simulink model "twin_numerico"  (R2024b)
settings: Solver=ode4  StartTime=0.0  StopTime=20  FixedStep=2e-4  RelTol=1e-3
InitFcn:
  | parameters_charlton;
  | parameters_chamber1d;
  | parameters_ferreira;
  | KT = 1.44; Tmax = KT*Tmax;
  | Emax = 1.40;
  | LAP = 8.50;
undefined symbols (not defined in the file): AP_0, C3, Emin, Ferreira_LV, L, MCL_vascular_lib, P_venous, R1, R2, R3, R4, S_abdominal, S_lower, S_upper, tc, V0, z1_0
settings Model: Creator=sammy  LastModifiedBy=sammy

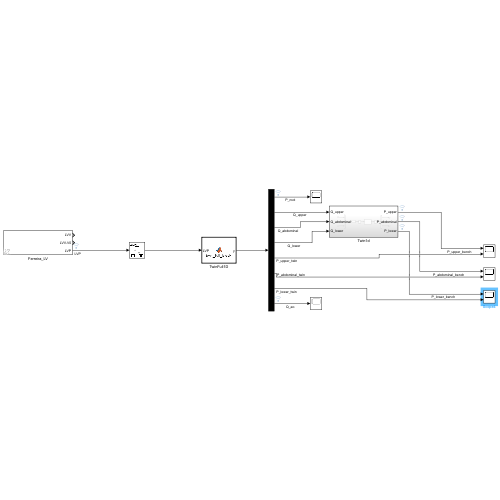
[thumbnail: Simulink's stored preview of the top-level diagram]
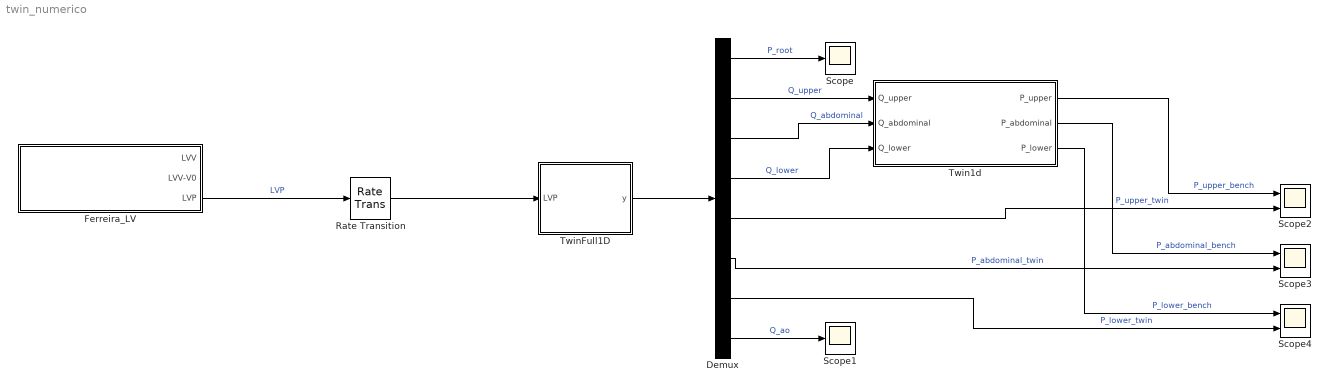
== system twin_numerico ==
  Demux : Demux  Outputs=8
  Ferreira_LV : Subsystem  AncestorBlock=MCL_vascular_lib/Ferreira_LV
  Rate Transition : RateTransition  OutPortSampleTime=1e-3
  Scope : Scope
  Scope1 : Scope
  Scope2 : Scope  NumInputPorts=2
  Scope3 : Scope  NumInputPorts=2
  Scope4 : Scope  NumInputPorts=2
  Twin1d : Subsystem
  TwinFull1D : MATLAB Function  TreatAsAtomicUnit=on
  wires:
  Ferreira_LV/3(LVP) -> Rate Transition/1  "LVP"
  Rate Transition/1 -> TwinFull1D/1(LVP)
  TwinFull1D/1(y) -> Demux/1
  Demux/1 -> Scope/1  "P_root"
  Demux/8 -> Scope1/1  "Q_ao"
  Demux/2 -> Twin1d/1(Q_upper)  "Q_upper"
  Demux/3 -> Twin1d/2(Q_abdominal)  "Q_abdominal"
  Demux/4 -> Twin1d/3(Q_lower)  "Q_lower"
  Demux/5 -> Scope2/2  "P_upper_twin"
  Demux/6 -> Scope3/2  "P_abdominal_twin"
  Demux/7 -> Scope4/2  "P_lower_twin"
  Twin1d/1(P_upper) -> Scope2/1  "P_upper_bench"
  Twin1d/2(P_abdominal) -> Scope3/1  "P_abdominal_bench"
  Twin1d/3(P_lower) -> Scope4/1  "P_lower_bench"

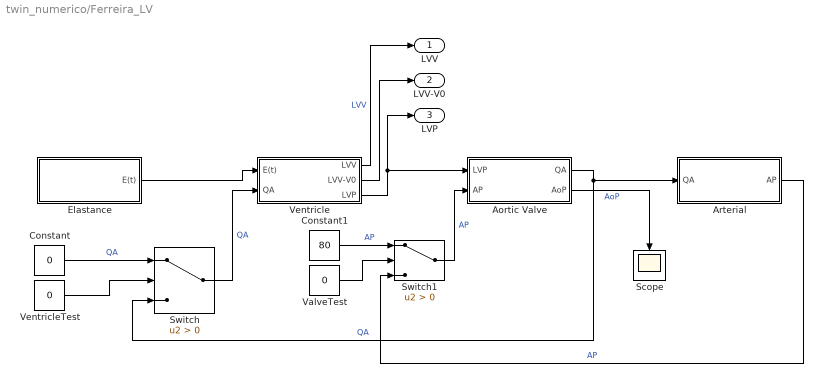
== system twin_numerico/Ferreira_LV ==
  Aortic Valve : Subsystem
  Arterial : Subsystem
  Constant : Constant  Value=0
  Constant1 : Constant  Value=80
  Elastance : Subsystem
  Scope : Scope
  Switch : Switch  Criteria=u2 > Threshold  SaturateOnIntegerOverflow=off  InputSameDT=off
  Switch1 : Switch  Criteria=u2 > Threshold  SaturateOnIntegerOverflow=off  InputSameDT=off
  ValveTest : Constant  Value=0
  Ventricle : Subsystem
  VentricleTest : Constant  Value=0
  LVV : Outport
  LVV-V0 : Outport  Port=2
  LVP : Outport  Port=3
  wires:
  VentricleTest/1 -> Switch/2
  Aortic Valve/1(QA) -> Arterial/1(QA), Switch/3  "QA"
  Ventricle/2(LVV-V0) -> LVV-V0/1
  Elastance/1(E(t)) -> Ventricle/1(E(t))
  Constant/1 -> Switch/1  "QA"
  Constant1/1 -> Switch1/1  "AP"
  Ventricle/3(LVP) -> LVP/1, Aortic Valve/1(LVP)
  Arterial/1(AP) -> Switch1/3  "AP"
  Switch/1 -> Ventricle/2(QA)  "QA"
  ValveTest/1 -> Switch1/2
  Switch1/1 -> Aortic Valve/2(AP)  "AP"
  Ventricle/1(LVV) -> LVV/1  "LVV"
  Aortic Valve/2(AoP) -> Scope/1  "AoP"

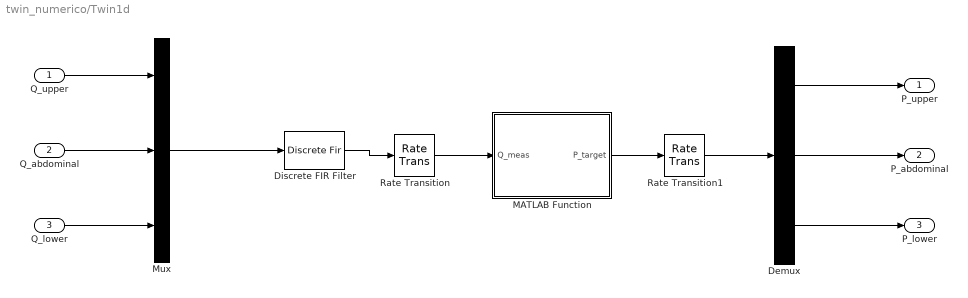
== system twin_numerico/Twin1d ==
  Q_upper : Inport
  Q_abdominal : Inport  Port=2
  Q_lower : Inport  Port=3
  Demux : Demux  Outputs=3
  Discrete FIR Filter : DiscreteFir  Coefficients=ones(1,5)/5
  MATLAB Function : MATLAB Function  TreatAsAtomicUnit=on
  Mux : Mux  Inputs=3
  Rate Transition : RateTransition  OutPortSampleTime=1e-3
  Rate Transition1 : RateTransition  OutPortSampleTime=2e-4
  P_upper : Outport
  P_abdominal : Outport  Port=2
  P_lower : Outport  Port=3
  wires:
  Q_upper/1 -> Mux/1
  Q_abdominal/1 -> Mux/2
  Q_lower/1 -> Mux/3
  Mux/1 -> Discrete FIR Filter/1
  Discrete FIR Filter/1 -> Rate Transition/1
  Rate Transition/1 -> MATLAB Function/1(Q_meas)
  MATLAB Function/1(P_target) -> Rate Transition1/1
  Rate Transition1/1 -> Demux/1
  Demux/1 -> P_upper/1
  Demux/2 -> P_abdominal/1
  Demux/3 -> P_lower/1

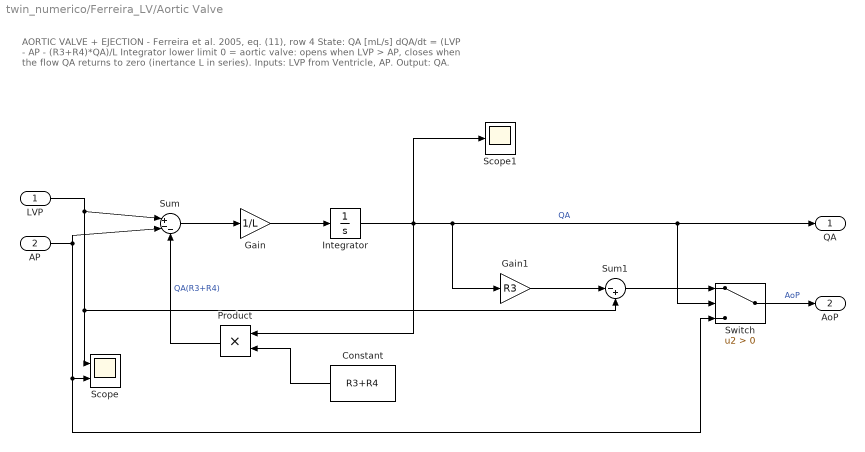
== system twin_numerico/Ferreira_LV/Aortic Valve ==
  note: AORTIC VALVE + EJECTION - Ferreira et al. 2005, eq. (11), row 4
      | State: QA [mL/s] dQA/dt = (LVP - AP - (R3+R4)*QA)/L
      | Integrator lower limit 0 = aortic valve: opens when LVP > AP, closes when the flow QA returns to zero (inertance L in series).
      | Inputs: LVP from Ventricle, AP. Output: QA.
  LVP : Inport
  AP : Inport  Port=2
  Constant : Constant  Value=R3+R4
  Gain : Gain  Gain=1/L
  Gain1 : Gain  Gain=R3
  Integrator : Integrator  LimitOutput=on  LowerSaturationLimit=0
  Product : Product
  Scope : Scope  NumInputPorts=2
  Scope1 : Scope
  Sum : Sum  Inputs=|+--
  Sum1 : Sum  Inputs=|-+
  Switch : Switch  Criteria=u2 > Threshold  SaturateOnIntegerOverflow=off  InputSameDT=off
  QA : Outport
  AoP : Outport  Port=2
  wires:
  LVP/1 -> Sum1/2, Scope/1, Sum/1
  AP/1 -> Switch/3, Scope/2, Sum/2
  Integrator/1 -> Scope1/1, Gain1/1, Switch/2, QA/1, Product/1  "QA"
  Constant/1 -> Product/2
  Product/1 -> Sum/3  "QA(R3+R4)"
  Sum/1 -> Gain/1
  Gain/1 -> Integrator/1
  Gain1/1 -> Sum1/1
  Sum1/1 -> Switch/1
  Switch/1 -> AoP/1  "AoP"

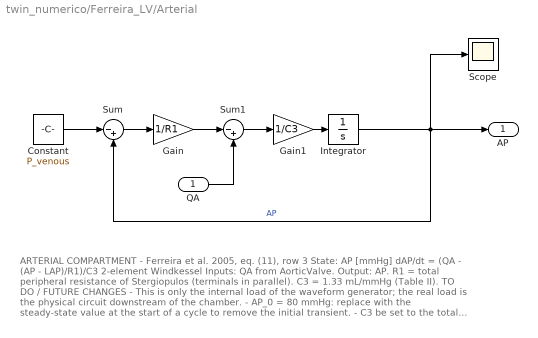
== system twin_numerico/Ferreira_LV/Arterial ==
  note: ARTERIAL COMPARTMENT - Ferreira et al. 2005, eq. (11), row 3
      | State: AP [mmHg] dAP/dt = (QA - (AP - LAP)/R1)/C3 2-element Windkessel
      | Inputs: QA from AorticValve. Output: AP. R1 = total peripheral resistance of Stergiopulos (terminals in parallel). C3 = 1.33 mL/mmHg (Table II).
      | TO DO / FUTURE CHANGES
      | - This is only the internal load of the waveform generator; the real load is the physical circuit downstream of the chamber.
      | - AP_0 = 80 mmHg: replace with the steady-state value at the start of a cycle to remove the initial transient.
      | - C3 be set to the total compliance of the Stergiopulos model for consistency with R1
  QA : Inport
  Constant : Constant  Value=P_venous
  Gain : Gain  Gain=1/R1
  Gain1 : Gain  Gain=1/C3
  Integrator : Integrator  InitialCondition=AP_0
  Scope : Scope
  Sum : Sum  Inputs=|-+
  Sum1 : Sum  Inputs=|-+
  AP : Outport
  wires:
  Constant/1 -> Sum/1
  Integrator/1 -> Scope/1, AP/1, Sum/2  "AP"
  Sum/1 -> Gain/1
  Gain/1 -> Sum1/1
  QA/1 -> Sum1/2
  Sum1/1 -> Gain1/1
  Gain1/1 -> Integrator/1

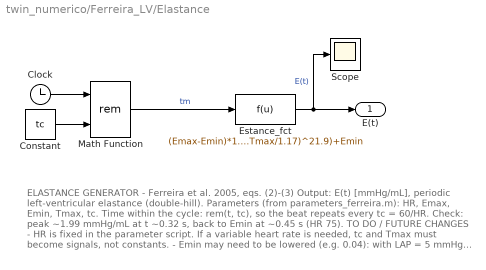
== system twin_numerico/Ferreira_LV/Elastance ==
  note: ELASTANCE GENERATOR - Ferreira et al. 2005, eqs. (2)-(3)
      | Output: E(t) [mmHg/mL], periodic left-ventricular elastance (double-hill).
      | Parameters (from parameters_ferreira.m):
      | HR, Emax, Emin, Tmax, tc.
      | Time within the cycle: rem(t, tc), so the beat repeats every tc = 60/HR.
      | Check: peak ~1.99 mmHg/mL at t ~0.32 s, back to Emin at ~0.45 s (HR 75).
      | TO DO / FUTURE CHANGES
      | - HR is fixed in the parameter script. If a variable heart rate is needed, tc and Tmax must become signals, not constants.
      | - Emin may need to be lowered (e.g. 0.04): with LAP = 5 mmHg the ventricle fills only to z1 = LAP/Emin ~ 83 mL (low stroke volume).
  Clock : Clock
  Constant : Constant  Value=tc
  Estance_fct : Fcn  Expr=(Emax-Emin)*1.55*((u/Tmax/0.7)^1.9/(1+(u/Tmax/0.7)^1.9))/(1+(u/Tmax/1.17)^21.9)+Emin
  Math Function : Math  Operator=rem
  Scope : Scope
  E(t) : Outport
  wires:
  Clock/1 -> Math Function/1
  Math Function/1 -> Estance_fct/1  "tm"
  Constant/1 -> Math Function/2
  Estance_fct/1 -> Scope/1, E(t)/1  "E(t)"

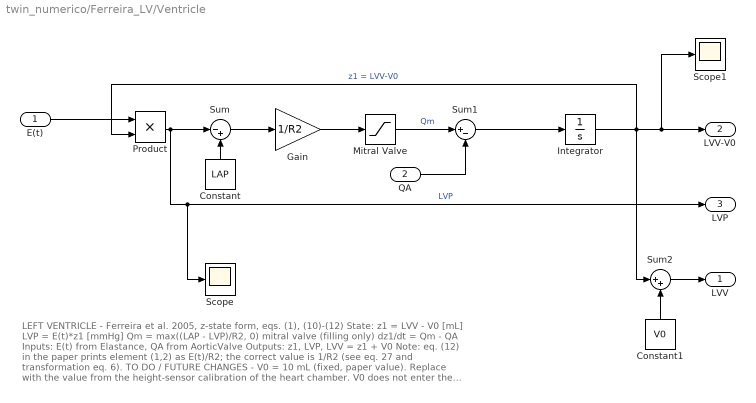
== system twin_numerico/Ferreira_LV/Ventricle ==
  note: LEFT VENTRICLE - Ferreira et al. 2005, z-state form, eqs. (1), (10)-(12)
      | State: z1 = LVV - V0 [mL] LVP = E(t)*z1 [mmHg] Qm = max((LAP - LVP)/R2, 0) mitral valve (filling only) dz1/dt = Qm - QA
      | Inputs: E(t) from Elastance, QA from AorticValve
      | Outputs: z1, LVP, LVV = z1 + V0
      | Note: eq. (12) in the paper prints element (1,2) as E(t)/R2; the correct value is 1/R2 (see eq. 27 and transformation eq. 6).
      | TO DO / FUTURE CHANGES
      | - V0 = 10 mL (fixed, paper value). Replace with the value from the height-sensor calibration of the heart chamber. V0 does not enter the dynamics, only the output LVV = z1 + V0. - LAP = P_venous (5 mmHg, constant), taken from parameters_stergiopulos.m. . - The output used by the physical chamber is the volume (LVV or z1); the conversion to pressure / chamber command is done outside this block.
  E(t) : Inport
  QA : Inport  Port=2
  Constant : Constant  Value=LAP
  Constant1 : Constant  Value=V0
  Gain : Gain  Gain=1/R2
  Integrator : Integrator  InitialCondition=z1_0
  Mitral Valve : Saturate  UpperLimit=inf  LowerLimit=0
  Product : Product
  Scope : Scope
  Scope1 : Scope
  Sum : Sum  Inputs=|-+
  Sum1 : Sum  Inputs=|+-
  Sum2 : Sum  Inputs=|++
  LVV : Outport
  LVV-V0 : Outport  Port=2
  LVP : Outport  Port=3
  wires:
  E(t)/1 -> Product/1
  Integrator/1 -> Sum2/1, Scope1/1, LVV-V0/1, Product/2  "z1 = LVV-V0"
  Product/1 -> Scope/1, LVP/1, Sum/1  "LVP"
  Constant/1 -> Sum/2
  Sum/1 -> Gain/1
  Gain/1 -> Mitral Valve/1
  Mitral Valve/1 -> Sum1/1  "Qm"
  QA/1 -> Sum1/2
  Sum1/1 -> Integrator/1
  Constant1/1 -> Sum2/2
  Sum2/1 -> LVV/1

== matlab function twin_numerico/Twin1d/MATLAB Function ==
  data: Q_meas input; P_target output; S_upper parameter; S_abdominal parameter; S_lower parameter
function P_target = twin_chambers_block(Q_meas, S_upper, S_abdominal, S_lower)
%TWIN_CHAMBERS_BLOCK  Body of the MATLAB Function block "Twin1D".
%   One block for the three Windkessel chambers.
%   Q_meas   [mL/s] 3x1 flow measured INTO each chamber (positive entering):
%                   [upper; abdominal; lower]
%   S_upper, S_abdominal, S_lower: 1D sub-trees from parameters_chamber1d.m,
%                   NON-TUNABLE parameters of the block
%   P_target [mmHg] 3x1 pressure each chamber must reproduce
%   Block sample time 1e-3 s (= S_*.dt), one solver step per call.
%#codegen
persistent Au Qu Pnu Pcu  Aa Qa Pna Pca  Al Ql Pnl Pcl
if isempty(Au)                                  % rest at P = DBP
    Au = S_upper.A0;      Qu = zeros(S_upper.nF,1);
    Pnu = S_upper.Pref*ones(S_upper.nNodes,1);      Pcu = S_upper.Pref*ones(numel(S_upper.tSeg),1);
    Aa = S_abdominal.A0;  Qa = zeros(S_abdominal.nF,1);
    Pna = S_abdominal.Pref*ones(S_abdominal.nNodes,1); Pca = S_abdominal.Pref*ones(numel(S_abdominal.tSeg),1);
    Al = S_lower.A0;      Ql = zeros(S_lower.nF,1);
    Pnl = S_lower.Pref*ones(S_lower.nNodes,1);      Pcl = S_lower.Pref*ones(numel(S_lower.tSeg),1);
end
[Au, Qu, Pnu, Pcu] = charlton1d_step(S_upper,     Au, Qu, Pnu, Pcu, 1e-6*Q_meas(1));
[Aa, Qa, Pna, Pca] = charlton1d_step(S_abdominal, Aa, Qa, Pna, Pca, 1e-6*Q_meas(2));
[Al, Ql, Pnl, Pcl] = charlton1d_step(S_lower,     Al, Ql, Pnl, Pcl, 1e-6*Q_meas(3));
P_target = [Pnu(S_upper.root); Pna(S_abdominal.root); Pnl(S_lower.root)]/133.322;
end

== matlab function twin_numerico/TwinFull1D ==
  settings: updateMethod=DISCRETE  sampleTime=1e-3
  data: LVP input; y output; S_full parameter
function y = twin_full_block(LVP, S_full)

%TWIN_FULL_BLOCK  Body of the MATLAB Function block "TwinFull1D": the whole
%   PWDB network (aorta of Charlton + upper, abdominal and lower trees).
%   LVP   [mmHg]  left-ventricular pressure (Ferreira generator), upstream of the valve
%   y     8x1:    [P_root; Q_upper; Q_abdominal; Q_lower; P_upper; P_abdominal; P_lower; Q_ao]
%   S_full        full network from parameters_chamber1d.m, NON-TUNABLE parameter
%   Block sample time 1e-3 s (= S_full.dt).
%#codegen
persistent A Q Pn Pc
if isempty(A)                                   % rest at P = DBP
    A  = S_full.A0;  Q = zeros(S_full.nF,1);
    Pn = S_full.Pref*ones(S_full.nNodes,1);  Pc = S_full.Pref*ones(numel(S_full.tSeg),1);
end
[A, Q, Pn, Pc, Qv] = charlton1d_step(S_full, A, Q, Pn, Pc, 0, ...
                                     LVP*133.322, S_full.Rv);
y = zeros(8,1);
y(1) = Pn(S_full.root)/133.322;
y(2) = 1e6*sum(Q(S_full.fUp));
y(3) = 1e6*sum(Q(S_full.fAb));
y(4) = 1e6*sum(Q(S_full.fLo));
y(5) = mean(cellP(S_full, A, S_full.cUp));
y(6) = mean(cellP(S_full, A, S_full.cAb));
y(7) = mean(cellP(S_full, A, S_full.cLo));
y(8) = 1e6*Qv;                                   % [mL/s]
end

function p = cellP(S, A, c)                     % [mmHg] elastic pressure in cells c
p = (S.Pref + S.beta(c)./S.A0(c).*(sqrt(A(c)) - S.sqA0(c)))/133.322;
end
